simulink library "Linkage"  (R2025b)
settings: Solver=VariableStepAuto  StartTime=0.0  StopTime=10.0  RelTol=1e-3
undefined symbols (not defined in the file): Axle1D, AxleIn, Chassis, Init, RaceFix, RaceSpin, Vehicle, Visual, X, Y, Z
libraries: sm_lib x940, nesl_utility x136, fl_lib x6, Linkage_Systems x2, SteeringWheel x2, Linkage_Decoupled x2, AntiRollBar_Systems x1, Steer_Rack_None x1, Steer_Rack_WheelDrivenRack1UJoint x1
(part 4 of 25)

== system Linkage/Susp/Linkage Decoupled/RollHeave Decouple/HP Heave L ==
  note: Shock point is not mirrored to permit independent point definition on left and right sides.
  note: Aligns pivot axis with vector normal to three hardpoints.
  Revolute Pivot : sm_lib/Joints/Revolute Joint  JointMode=Normal  CompositeWrenchDir=FollowerOnBase  CompositeWrenchFrame=BaseFrame  SenseConstraintForce=off  SenseConstraintTorque=off  SenseTotalForce=off  SenseTotalTorque=off  PositionTargetSpecify=off  PositionTargetPriority=Low  PositionTargetValue=0  PositionTargetValueUnits=deg  VelocityTargetSpecify=off  VelocityTargetPriority=High  VelocityTargetValue=0  VelocityTargetValueUnits=deg/s  EquilibriumPosition=0  EquilibriumPositionUnits=deg  SpringStiffness=0  SpringStiffnessUnits=N*m/deg  DampingCoefficient=0  DampingCoefficientUnits=N*m/(deg/s)  LowerLimitSpecify=off  LowerLimitBound=-90  LowerLimitBoundUnits=deg  LowerLimitStiffness=1e4  LowerLimitStiffnessUnits=N*m/deg  LowerLimitDamping=10  LowerLimitDampingUnits=N*m/(deg/s)  LowerLimitTransitionRegionWidth=0.1  LowerLimitTransitionRegionWidthUnits=deg  UpperLimitSpecify=off  UpperLimitBound=90  UpperLimitBoundUnits=deg  UpperLimitStiffness=1e4  UpperLimitStiffnessUnits=N*m/deg  UpperLimitDamping=10  UpperLimitDampingUnits=N*m/(deg/s)  UpperLimitTransitionRegionWidth=0.1  UpperLimitTransitionRegionWidthUnits=deg  TorqueActuationMode=NoTorque  MotionActuationMode=ComputedMotion  SensePosition=on  SenseVelocity=off  SenseAcceleration=off  SenseTorqueForce=off  SenseLowerLimitTorqueForce=off  SenseUpperLimitTorqueForce=off
  Transform Align Axis B : Subsystem  mask(Transform Align Axis Three Points){pt1=hp_bcr_pivot.*rhs_hp, pt2=hp_pushrod_in.*rhs_hp, pt3=hp_bcr_shock, popup_f_axis=+Z}
      mask prompts: pt1 "Point 1 [xyz] (m)"; pt2 "Point 2 [xyz] (m)"; pt3 "Point 3 [xyz] (m)"; popup_f_axis "Axis of F Frame to Aim at Target"
      mask help: Transforms a frame to aim a selected axis along a normal to a plane defined by 3 points. All points must be defined relative to the same reference frame. Normal to the plane is defined as cross (HP1 -> HP3, HP1->HP2).
      mask init:
      | switch popup_f_axis
      |     case 1, vec = [ 1  0  0];
      |     case 2, vec = [ 0  1  0];
      |     case 3, vec = [ 0  0  1];
      |     case 4, vec = [-1  0  0];
      |     case 5, vec = [ 0 -1  0];
      |     case 6, vec = [ 0  0 -1];
      | end
      | 
      | % Unit vectors 
      | uvec1 = (pt3-pt1)/norm(pt3-pt1);
      | uvec2 = (pt2-pt1)/norm(pt2-pt1);
      | 
      | nvec = cross(uvec1,uvec2);
      | unvec = nvec/norm(nvec);
      | 
      | % Force nvec to point along +z
      | %if(unvec(3)<0)
      | %    unvec = -unvec;
      | %end
      | rotaxis = cross(vec,unvec);
      | 
      | if (norm(rotaxis)==0)
      |     if (sum(uvec1==0)==3 || sum(uvec2==0)==3)  % hps collocated
      |         rotangle = 0; 
      |     elseif ((sum(uvec1+uvec2)==0) ...  % vectors antiparallel    
      |             || (sum(vec+unvec))==0)    % vec and unvec antiparallel
      |         rotangle = pi;
      |         rotaxis = circshift(vec,1);
      |     else                       % vectors parallel
      |         rotangle = 0;          
      |     end
      | else
      |     rotangle = acos(dot(vec,unvec));
      |     %rotangle = acos(dot(vec,(hp_t-hp_b)/norm((hp_t-hp_b))))
      | end
      mask TypeOptions popup_f_axis: +X | +Y | +Z | -X | -Y | -Z
      mask Display: image('sm_car_transform_align_axis_three_points.png')
  Transform Align Axis F : Subsystem  mask(Transform Align Axis Three Points){pt1=hp_bcr_pivot.*rhs_hp, pt2=hp_pushrod_in.*rhs_hp, pt3=hp_bcr_shock, popup_f_axis=+Z}
      mask prompts: pt1 "Point 1 [xyz] (m)"; pt2 "Point 2 [xyz] (m)"; pt3 "Point 3 [xyz] (m)"; popup_f_axis "Axis of F Frame to Aim at Target"
      mask help: Transforms a frame to aim a selected axis along a normal to a plane defined by 3 points. All points must be defined relative to the same reference frame. Normal to the plane is defined as cross (HP1 -> HP3, HP1->HP2).
      mask init: same as Linkage/Susp/Linkage Decoupled/RollHeave Decouple/HP Heave L/Transform Align Axis B
      mask TypeOptions popup_f_axis: +X | +Y | +Z | -X | -Y | -Z
      mask Display: image('sm_car_transform_align_axis_three_points.png')
  F : PMIOPort  Side=Right
  B : PMIOPort  Port=2  Side=Left
  q : PMIOPort  Port=3  Side=Right
  connections:
  Transform Align Axis B/LConn1 -- B/RConn1
  Transform Align Axis F/RConn1 -- Revolute Pivot/RConn1
  Revolute Pivot/LConn1 -- Transform Align Axis B/RConn1
  Transform Align Axis F/LConn1 -- F/RConn1
  q/RConn1 -- Revolute Pivot/RConn2

== system Linkage/Susp/Linkage Decoupled/RollHeave Decouple/HP HeaveR ==
  note: Shock point is not mirrored to permit independent point definition on left and right sides.
  note: Aligns pivot axis with vector normal to three hardpoints.
  Revolute Pivot : sm_lib/Joints/Revolute Joint  JointMode=Normal  CompositeWrenchDir=FollowerOnBase  CompositeWrenchFrame=BaseFrame  SenseConstraintForce=off  SenseConstraintTorque=off  SenseTotalForce=off  SenseTotalTorque=off  PositionTargetSpecify=off  PositionTargetPriority=Low  PositionTargetValue=0  PositionTargetValueUnits=deg  VelocityTargetSpecify=off  VelocityTargetPriority=High  VelocityTargetValue=0  VelocityTargetValueUnits=deg/s  EquilibriumPosition=0  EquilibriumPositionUnits=deg  SpringStiffness=0  SpringStiffnessUnits=N*m/deg  DampingCoefficient=0  DampingCoefficientUnits=N*m/(deg/s)  LowerLimitSpecify=off  LowerLimitBound=-90  LowerLimitBoundUnits=deg  LowerLimitStiffness=1e4  LowerLimitStiffnessUnits=N*m/deg  LowerLimitDamping=10  LowerLimitDampingUnits=N*m/(deg/s)  LowerLimitTransitionRegionWidth=0.1  LowerLimitTransitionRegionWidthUnits=deg  UpperLimitSpecify=off  UpperLimitBound=90  UpperLimitBoundUnits=deg  UpperLimitStiffness=1e4  UpperLimitStiffnessUnits=N*m/deg  UpperLimitDamping=10  UpperLimitDampingUnits=N*m/(deg/s)  UpperLimitTransitionRegionWidth=0.1  UpperLimitTransitionRegionWidthUnits=deg  TorqueActuationMode=NoTorque  MotionActuationMode=ComputedMotion  SensePosition=on  SenseVelocity=off  SenseAcceleration=off  SenseTorqueForce=off  SenseLowerLimitTorqueForce=off  SenseUpperLimitTorqueForce=off
  Transform Align Axis B : Subsystem  mask(Transform Align Axis Three Points){pt1=hp_bcr_pivot.*rhs_hp, pt2=hp_pushrod_in.*rhs_hp, pt3=hp_bcr_shock, popup_f_axis=+Z}
      mask prompts: pt1 "Point 1 [xyz] (m)"; pt2 "Point 2 [xyz] (m)"; pt3 "Point 3 [xyz] (m)"; popup_f_axis "Axis of F Frame to Aim at Target"
      mask help: Transforms a frame to aim a selected axis along a normal to a plane defined by 3 points. All points must be defined relative to the same reference frame. Normal to the plane is defined as cross (HP1 -> HP3, HP1->HP2).
      mask init: same as Linkage/Susp/Linkage Decoupled/RollHeave Decouple/HP Heave L/Transform Align Axis B
      mask TypeOptions popup_f_axis: +X | +Y | +Z | -X | -Y | -Z
      mask Display: image('sm_car_transform_align_axis_three_points.png')
  Transform Align Axis F : Subsystem  mask(Transform Align Axis Three Points){pt1=hp_bcr_pivot.*rhs_hp, pt2=hp_pushrod_in.*rhs_hp, pt3=hp_bcr_shock, popup_f_axis=+Z}
      mask prompts: pt1 "Point 1 [xyz] (m)"; pt2 "Point 2 [xyz] (m)"; pt3 "Point 3 [xyz] (m)"; popup_f_axis "Axis of F Frame to Aim at Target"
      mask help: Transforms a frame to aim a selected axis along a normal to a plane defined by 3 points. All points must be defined relative to the same reference frame. Normal to the plane is defined as cross (HP1 -> HP3, HP1->HP2).
      mask init: same as Linkage/Susp/Linkage Decoupled/RollHeave Decouple/HP Heave L/Transform Align Axis B
      mask TypeOptions popup_f_axis: +X | +Y | +Z | -X | -Y | -Z
      mask Display: image('sm_car_transform_align_axis_three_points.png')
  F : PMIOPort  Side=Right
  B : PMIOPort  Port=2  Side=Left
  q : PMIOPort  Port=3  Side=Right
  connections:
  Transform Align Axis F/LConn1 -- F/RConn1
  Revolute Pivot/LConn1 -- Transform Align Axis B/RConn1
  Transform Align Axis F/RConn1 -- Revolute Pivot/RConn1
  Transform Align Axis B/LConn1 -- B/RConn1
  q/RConn1 -- Revolute Pivot/RConn2

== system Linkage/Susp/Linkage Decoupled/RollHeave Decouple/HP Roll L ==
  note: Shock point is not mirrored to permit independent point definition on left and right sides.
  note: Aligns pivot axis with vector normal to three hardpoints.
  Revolute Pivot : sm_lib/Joints/Revolute Joint  JointMode=Normal  CompositeWrenchDir=FollowerOnBase  CompositeWrenchFrame=BaseFrame  SenseConstraintForce=off  SenseConstraintTorque=off  SenseTotalForce=off  SenseTotalTorque=off  PositionTargetSpecify=off  PositionTargetPriority=Low  PositionTargetValue=0  PositionTargetValueUnits=deg  VelocityTargetSpecify=off  VelocityTargetPriority=High  VelocityTargetValue=0  VelocityTargetValueUnits=deg/s  EquilibriumPosition=0  EquilibriumPositionUnits=deg  SpringStiffness=0  SpringStiffnessUnits=N*m/deg  DampingCoefficient=0  DampingCoefficientUnits=N*m/(deg/s)  LowerLimitSpecify=off  LowerLimitBound=-90  LowerLimitBoundUnits=deg  LowerLimitStiffness=1e4  LowerLimitStiffnessUnits=N*m/deg  LowerLimitDamping=10  LowerLimitDampingUnits=N*m/(deg/s)  LowerLimitTransitionRegionWidth=0.1  LowerLimitTransitionRegionWidthUnits=deg  UpperLimitSpecify=off  UpperLimitBound=90  UpperLimitBoundUnits=deg  UpperLimitStiffness=1e4  UpperLimitStiffnessUnits=N*m/deg  UpperLimitDamping=10  UpperLimitDampingUnits=N*m/(deg/s)  UpperLimitTransitionRegionWidth=0.1  UpperLimitTransitionRegionWidthUnits=deg  TorqueActuationMode=NoTorque  MotionActuationMode=ComputedMotion  SensePosition=on  SenseVelocity=off  SenseAcceleration=off  SenseTorqueForce=off  SenseLowerLimitTorqueForce=off  SenseUpperLimitTorqueForce=off
  Transform Align Axis B : Subsystem  mask(Transform Align Axis Three Points){pt1=hp_bcr_pivot.*rhs_hp, pt2=hp_pushrod_in.*rhs_hp, pt3=hp_bcr_shock, popup_f_axis=+Z}
      mask prompts: pt1 "Point 1 [xyz] (m)"; pt2 "Point 2 [xyz] (m)"; pt3 "Point 3 [xyz] (m)"; popup_f_axis "Axis of F Frame to Aim at Target"
      mask help: Transforms a frame to aim a selected axis along a normal to a plane defined by 3 points. All points must be defined relative to the same reference frame. Normal to the plane is defined as cross (HP1 -> HP3, HP1->HP2).
      mask init: same as Linkage/Susp/Linkage Decoupled/RollHeave Decouple/HP Heave L/Transform Align Axis B
      mask TypeOptions popup_f_axis: +X | +Y | +Z | -X | -Y | -Z
      mask Display: image('sm_car_transform_align_axis_three_points.png')
  Transform Align Axis F : Subsystem  mask(Transform Align Axis Three Points){pt1=hp_bcr_pivot.*rhs_hp, pt2=hp_pushrod_in.*rhs_hp, pt3=hp_bcr_shock, popup_f_axis=+Z}
      mask prompts: pt1 "Point 1 [xyz] (m)"; pt2 "Point 2 [xyz] (m)"; pt3 "Point 3 [xyz] (m)"; popup_f_axis "Axis of F Frame to Aim at Target"
      mask help: Transforms a frame to aim a selected axis along a normal to a plane defined by 3 points. All points must be defined relative to the same reference frame. Normal to the plane is defined as cross (HP1 -> HP3, HP1->HP2).
      mask init: same as Linkage/Susp/Linkage Decoupled/RollHeave Decouple/HP Heave L/Transform Align Axis B
      mask TypeOptions popup_f_axis: +X | +Y | +Z | -X | -Y | -Z
      mask Display: image('sm_car_transform_align_axis_three_points.png')
  F : PMIOPort  Side=Right
  B : PMIOPort  Port=2  Side=Left
  q : PMIOPort  Port=3  Side=Right
  connections:
  Transform Align Axis F/LConn1 -- F/RConn1
  Revolute Pivot/LConn1 -- Transform Align Axis B/RConn1
  Transform Align Axis F/RConn1 -- Revolute Pivot/RConn1
  Transform Align Axis B/LConn1 -- B/RConn1
  q/RConn1 -- Revolute Pivot/RConn2

== system Linkage/Susp/Linkage Decoupled/RollHeave Decouple/HP Roll R ==
  note: Shock point is not mirrored to permit independent point definition on left and right sides.
  note: Aligns pivot axis with vector normal to three hardpoints.
  Revolute Pivot : sm_lib/Joints/Revolute Joint  JointMode=Normal  CompositeWrenchDir=FollowerOnBase  CompositeWrenchFrame=BaseFrame  SenseConstraintForce=off  SenseConstraintTorque=off  SenseTotalForce=off  SenseTotalTorque=off  PositionTargetSpecify=off  PositionTargetPriority=Low  PositionTargetValue=0  PositionTargetValueUnits=deg  VelocityTargetSpecify=off  VelocityTargetPriority=High  VelocityTargetValue=0  VelocityTargetValueUnits=deg/s  EquilibriumPosition=0  EquilibriumPositionUnits=deg  SpringStiffness=0  SpringStiffnessUnits=N*m/deg  DampingCoefficient=0  DampingCoefficientUnits=N*m/(deg/s)  LowerLimitSpecify=off  LowerLimitBound=-90  LowerLimitBoundUnits=deg  LowerLimitStiffness=1e4  LowerLimitStiffnessUnits=N*m/deg  LowerLimitDamping=10  LowerLimitDampingUnits=N*m/(deg/s)  LowerLimitTransitionRegionWidth=0.1  LowerLimitTransitionRegionWidthUnits=deg  UpperLimitSpecify=off  UpperLimitBound=90  UpperLimitBoundUnits=deg  UpperLimitStiffness=1e4  UpperLimitStiffnessUnits=N*m/deg  UpperLimitDamping=10  UpperLimitDampingUnits=N*m/(deg/s)  UpperLimitTransitionRegionWidth=0.1  UpperLimitTransitionRegionWidthUnits=deg  TorqueActuationMode=NoTorque  MotionActuationMode=ComputedMotion  SensePosition=on  SenseVelocity=off  SenseAcceleration=off  SenseTorqueForce=off  SenseLowerLimitTorqueForce=off  SenseUpperLimitTorqueForce=off
  Transform Align Axis B : Subsystem  mask(Transform Align Axis Three Points){pt1=hp_bcr_pivot.*rhs_hp, pt2=hp_pushrod_in.*rhs_hp, pt3=hp_bcr_shock, popup_f_axis=+Z}
      mask prompts: pt1 "Point 1 [xyz] (m)"; pt2 "Point 2 [xyz] (m)"; pt3 "Point 3 [xyz] (m)"; popup_f_axis "Axis of F Frame to Aim at Target"
      mask help: Transforms a frame to aim a selected axis along a normal to a plane defined by 3 points. All points must be defined relative to the same reference frame. Normal to the plane is defined as cross (HP1 -> HP3, HP1->HP2).
      mask init: same as Linkage/Susp/Linkage Decoupled/RollHeave Decouple/HP Heave L/Transform Align Axis B
      mask TypeOptions popup_f_axis: +X | +Y | +Z | -X | -Y | -Z
      mask Display: image('sm_car_transform_align_axis_three_points.png')
  Transform Align Axis F : Subsystem  mask(Transform Align Axis Three Points){pt1=hp_bcr_pivot.*rhs_hp, pt2=hp_pushrod_in.*rhs_hp, pt3=hp_bcr_shock, popup_f_axis=+Z}
      mask prompts: pt1 "Point 1 [xyz] (m)"; pt2 "Point 2 [xyz] (m)"; pt3 "Point 3 [xyz] (m)"; popup_f_axis "Axis of F Frame to Aim at Target"
      mask help: Transforms a frame to aim a selected axis along a normal to a plane defined by 3 points. All points must be defined relative to the same reference frame. Normal to the plane is defined as cross (HP1 -> HP3, HP1->HP2).
      mask init: same as Linkage/Susp/Linkage Decoupled/RollHeave Decouple/HP Heave L/Transform Align Axis B
      mask TypeOptions popup_f_axis: +X | +Y | +Z | -X | -Y | -Z
      mask Display: image('sm_car_transform_align_axis_three_points.png')
  F : PMIOPort  Side=Right
  B : PMIOPort  Port=2  Side=Left
  q : PMIOPort  Port=3  Side=Right
  connections:
  Transform Align Axis B/LConn1 -- B/RConn1
  Transform Align Axis F/RConn1 -- Revolute Pivot/RConn1
  Revolute Pivot/LConn1 -- Transform Align Axis B/RConn1
  Transform Align Axis F/LConn1 -- F/RConn1
  q/RConn1 -- Revolute Pivot/RConn2

== system Linkage/Susp/Linkage Decoupled/RollHeave Decouple/Shock Heave ==
  Cylinder : Subsystem
  MTRef : fl_lib/Mechanical/Translational Elements/Mechanical Translational Reference
  PS-Simulink Converter : nesl_utility/PS-Simulink Converter  PhysicalDomain=network_engine_domain  SubClassName=ps_output  LeftPortType=input  RightPortType=output  PseudoPeriodic=off  Frequencies=[]  VectorFormat=1-D array  Unit=1  AffineConversion=off
  Piston : Subsystem
  Prismatic Spring : sm_lib/Joints/Prismatic Joint  JointMode=Normal  CompositeWrenchDir=FollowerOnBase  CompositeWrenchFrame=BaseFrame  SenseConstraintForce=off  SenseConstraintTorque=off  SenseTotalForce=off  SenseTotalTorque=off  PositionTargetSpecify=on  PositionTargetPriority=High  PositionTargetValue=init_spr_len  PositionTargetValueUnits=m  VelocityTargetSpecify=off  VelocityTargetPriority=High  VelocityTargetValue=0  VelocityTargetValueUnits=m/s  EquilibriumPosition=0  EquilibriumPositionUnits=m  SpringStiffness=0  SpringStiffnessUnits=N/m  DampingCoefficient=0.01  DampingCoefficientUnits=N/(m/s)  LowerLimitSpecify=off  LowerLimitBound=-1  LowerLimitBoundUnits=m  LowerLimitStiffness=1e6  LowerLimitStiffnessUnits=N/m  LowerLimitDamping=1e3  LowerLimitDampingUnits=N/(m/s)  LowerLimitTransitionRegionWidth=1e-4  LowerLimitTransitionRegionWidthUnits=m  UpperLimitSpecify=off  UpperLimitBound=1  UpperLimitBoundUnits=m  UpperLimitStiffness=1e6  UpperLimitStiffnessUnits=N/m  UpperLimitDamping=1e3  UpperLimitDampingUnits=N/(m/s)  UpperLimitTransitionRegionWidth=1e-4  UpperLimitTransitionRegionWidthUnits=m  TorqueActuationMode=InputTorque  MotionActuationMode=ComputedMotion  SensePosition=on  SenseVelocity=on  SenseAcceleration=off  SenseTorqueForce=off  SenseLowerLimitTorqueForce=off  SenseUpperLimitTorqueForce=off
  Translational Simscape Intf : Subsystem
  Vis HP L : sm_lib/Body Elements/Spherical Solid  SphereRadius=size_conn_shock  SphereRadiusUnits=m  ExportEntireGeometry=off  InertiaType=PointMass  BasedOnType=Density  Density=0  DensityUnits=kg/m^3  Mass=0  MassUnits=kg  CenterOfMass=[0 0 0]  CenterOfMassUnits=m  MomentsOfInertia=[1 1 1]  MomentsOfInertiaUnits=kg*m^2  ProductsOfInertia=[0 0 0]  ProductsOfInertiaUnits=kg*m^2  GraphicType=FromGeometry  MarkerShape=Sphere  MarkerSize=10  GraphicVisPropType=SimpleVisualProperties  GraphicDiffuseColor=clr_conn_shock  GraphicOpacity=opc_conn_shock  GraphicSpecularColor=[0.5 0.5 0.5 1.0]  GraphicAmbientColor=[0.15 0.15 0.15 1.0]  GraphicEmissiveColor=[0.0 0.0 0.0 1.0]  GraphicShininess=75  DoExposeReferenceFrame=on  SerializedFrames=<Frames/>
  Vis HP U : sm_lib/Body Elements/Spherical Solid  SphereRadius=size_conn_shock  SphereRadiusUnits=m  ExportEntireGeometry=off  InertiaType=PointMass  BasedOnType=Density  Density=0  DensityUnits=kg/m^3  Mass=0  MassUnits=kg  CenterOfMass=[0 0 0]  CenterOfMassUnits=m  MomentsOfInertia=[1 1 1]  MomentsOfInertiaUnits=kg*m^2  ProductsOfInertia=[0 0 0]  ProductsOfInertiaUnits=kg*m^2  GraphicType=FromGeometry  MarkerShape=Sphere  MarkerSize=10  GraphicVisPropType=SimpleVisualProperties  GraphicDiffuseColor=clr_conn_shock  GraphicOpacity=opc_conn_shock  GraphicSpecularColor=[0.5 0.5 0.5 1.0]  GraphicAmbientColor=[0.15 0.15 0.15 1.0]  GraphicEmissiveColor=[0.0 0.0 0.0 1.0]  GraphicShininess=75  DoExposeReferenceFrame=on  SerializedFrames=<Frames/>
  R : PMIOPort  Side=Right
  U : PMIOPort  Port=2  Side=Right
  L : PMIOPort  Port=3  Side=Left
  Out Bus Element : Outport  VectorParamsAs1DForOutWhenUnconnected=off  PortName=m  Element=x
  wires:
  PS-Simulink Converter/1 -> Out Bus Element/1
  connections:
  PS-Simulink Converter/LConn1 -- Prismatic Spring/RConn2
  Vis HP L/RConn1 -- Cylinder/LConn1 -- Prismatic Spring/LConn1 -- L/RConn1
  Translational Simscape Intf/LConn1 -- Prismatic Spring/LConn2
  Translational Simscape Intf/RConn1 -- Prismatic Spring/RConn3
  Vis HP U/RConn1 -- U/RConn1 -- Prismatic Spring/RConn1 -- Piston/RConn1
  MTRef/LConn1 -- Translational Simscape Intf/LConn2
  R/RConn1 -- Translational Simscape Intf/RConn2

== system Linkage/Susp/Linkage Decoupled/RollHeave Decouple/Shock Roll ==
  Cylinder : Subsystem
  MTRef : fl_lib/Mechanical/Translational Elements/Mechanical Translational Reference
  PS-Simulink Converter : nesl_utility/PS-Simulink Converter  PhysicalDomain=network_engine_domain  SubClassName=ps_output  LeftPortType=input  RightPortType=output  PseudoPeriodic=off  Frequencies=[]  VectorFormat=1-D array  Unit=1  AffineConversion=off
  Piston : Subsystem
  Prismatic Spring : sm_lib/Joints/Prismatic Joint  JointMode=Normal  CompositeWrenchDir=FollowerOnBase  CompositeWrenchFrame=BaseFrame  SenseConstraintForce=off  SenseConstraintTorque=off  SenseTotalForce=off  SenseTotalTorque=off  PositionTargetSpecify=on  PositionTargetPriority=High  PositionTargetValue=init_spr_len  PositionTargetValueUnits=m  VelocityTargetSpecify=off  VelocityTargetPriority=High  VelocityTargetValue=0  VelocityTargetValueUnits=m/s  EquilibriumPosition=0  EquilibriumPositionUnits=m  SpringStiffness=0  SpringStiffnessUnits=N/m  DampingCoefficient=0.01  DampingCoefficientUnits=N/(m/s)  LowerLimitSpecify=off  LowerLimitBound=-1  LowerLimitBoundUnits=m  LowerLimitStiffness=1e6  LowerLimitStiffnessUnits=N/m  LowerLimitDamping=1e3  LowerLimitDampingUnits=N/(m/s)  LowerLimitTransitionRegionWidth=1e-4  LowerLimitTransitionRegionWidthUnits=m  UpperLimitSpecify=off  UpperLimitBound=1  UpperLimitBoundUnits=m  UpperLimitStiffness=1e6  UpperLimitStiffnessUnits=N/m  UpperLimitDamping=1e3  UpperLimitDampingUnits=N/(m/s)  UpperLimitTransitionRegionWidth=1e-4  UpperLimitTransitionRegionWidthUnits=m  TorqueActuationMode=InputTorque  MotionActuationMode=ComputedMotion  SensePosition=on  SenseVelocity=on  SenseAcceleration=off  SenseTorqueForce=off  SenseLowerLimitTorqueForce=off  SenseUpperLimitTorqueForce=off
  Translational Simscape Intf : Subsystem
  Vis HP L : sm_lib/Body Elements/Spherical Solid  SphereRadius=size_conn_shock  SphereRadiusUnits=m  ExportEntireGeometry=off  InertiaType=PointMass  BasedOnType=Density  Density=0  DensityUnits=kg/m^3  Mass=0  MassUnits=kg  CenterOfMass=[0 0 0]  CenterOfMassUnits=m  MomentsOfInertia=[1 1 1]  MomentsOfInertiaUnits=kg*m^2  ProductsOfInertia=[0 0 0]  ProductsOfInertiaUnits=kg*m^2  GraphicType=FromGeometry  MarkerShape=Sphere  MarkerSize=10  GraphicVisPropType=SimpleVisualProperties  GraphicDiffuseColor=clr_conn_shock  GraphicOpacity=opc_conn_shock  GraphicSpecularColor=[0.5 0.5 0.5 1.0]  GraphicAmbientColor=[0.15 0.15 0.15 1.0]  GraphicEmissiveColor=[0.0 0.0 0.0 1.0]  GraphicShininess=75  DoExposeReferenceFrame=on  SerializedFrames=<Frames/>
  Vis HP U : sm_lib/Body Elements/Spherical Solid  SphereRadius=size_conn_shock  SphereRadiusUnits=m  ExportEntireGeometry=off  InertiaType=PointMass  BasedOnType=Density  Density=0  DensityUnits=kg/m^3  Mass=0  MassUnits=kg  CenterOfMass=[0 0 0]  CenterOfMassUnits=m  MomentsOfInertia=[1 1 1]  MomentsOfInertiaUnits=kg*m^2  ProductsOfInertia=[0 0 0]  ProductsOfInertiaUnits=kg*m^2  GraphicType=FromGeometry  MarkerShape=Sphere  MarkerSize=10  GraphicVisPropType=SimpleVisualProperties  GraphicDiffuseColor=clr_conn_shock  GraphicOpacity=opc_conn_shock  GraphicSpecularColor=[0.5 0.5 0.5 1.0]  GraphicAmbientColor=[0.15 0.15 0.15 1.0]  GraphicEmissiveColor=[0.0 0.0 0.0 1.0]  GraphicShininess=75  DoExposeReferenceFrame=on  SerializedFrames=<Frames/>
  R : PMIOPort  Side=Right
  U : PMIOPort  Port=2  Side=Right
  L : PMIOPort  Port=3  Side=Left
  Out Bus Element : Outport  VectorParamsAs1DForOutWhenUnconnected=off  PortName=m  Element=x
  wires:
  PS-Simulink Converter/1 -> Out Bus Element/1
  connections:
  PS-Simulink Converter/LConn1 -- Prismatic Spring/RConn2
  Vis HP L/RConn1 -- Cylinder/LConn1 -- Prismatic Spring/LConn1 -- L/RConn1
  Translational Simscape Intf/LConn1 -- Prismatic Spring/LConn2
  Translational Simscape Intf/RConn1 -- Prismatic Spring/RConn3
  Vis HP U/RConn1 -- U/RConn1 -- Prismatic Spring/RConn1 -- Piston/RConn1
  MTRef/LConn1 -- Translational Simscape Intf/LConn2
  R/RConn1 -- Translational Simscape Intf/RConn2

== system Linkage/Susp/Linkage Decoupled/RollHeave Decouple/Transform Align Axis 2P HeaveL ==
  Transform : sm_lib/Frames and Transforms/Rigid Transform  RotationMethod=ArbitraryAxis  FollAlignAxisA=+X  BaseAlignAxisA=+Y  FollAlignAxisB=+Y  BaseAlignAxisB=+Z  RotationStandardAxis=+Z  RotationAngle=rotangle  RotationAngleUnits=rad  RotationArbitraryAxis=rotaxis  RotationSequenceAxes=FollowerAxes  RotationSequence=XYX  RotationSequenceAngles=[0 0 0]  RotationSequenceAnglesUnits=deg  RotationMatrix=[1 0 0; 0 1 0; 0 0 1]  Quaternion=[1 0 0 0]  TranslationMethod=None  TranslationCartesianOffset=[0 0 0]  TranslationCartesianOffsetUnits=m  TranslationStandardAxis=+Z  TranslationStandardOffset=0  TranslationStandardOffsetUnits=m  TranslationROffset=0  TranslationROffsetUnits=m  TranslationThetaOffset=0  TranslationThetaOffsetUnits=deg  TranslationZOffset=0  TranslationZOffsetUnits=m
  B : PMIOPort  Side=Left
  F : PMIOPort  Port=2  Side=Right
  connections:
  Transform/LConn1 -- B/RConn1
  Transform/RConn1 -- F/RConn1

== system Linkage/Susp/Linkage Decoupled/RollHeave Decouple/Transform Align Axis 2P HeaveR ==
  Transform : sm_lib/Frames and Transforms/Rigid Transform  RotationMethod=ArbitraryAxis  FollAlignAxisA=+X  BaseAlignAxisA=+Y  FollAlignAxisB=+Y  BaseAlignAxisB=+Z  RotationStandardAxis=+Z  RotationAngle=rotangle  RotationAngleUnits=rad  RotationArbitraryAxis=rotaxis  RotationSequenceAxes=FollowerAxes  RotationSequence=XYX  RotationSequenceAngles=[0 0 0]  RotationSequenceAnglesUnits=deg  RotationMatrix=[1 0 0; 0 1 0; 0 0 1]  Quaternion=[1 0 0 0]  TranslationMethod=None  TranslationCartesianOffset=[0 0 0]  TranslationCartesianOffsetUnits=m  TranslationStandardAxis=+Z  TranslationStandardOffset=0  TranslationStandardOffsetUnits=m  TranslationROffset=0  TranslationROffsetUnits=m  TranslationThetaOffset=0  TranslationThetaOffsetUnits=deg  TranslationZOffset=0  TranslationZOffsetUnits=m
  B : PMIOPort  Side=Left
  F : PMIOPort  Port=2  Side=Right
  connections:
  Transform/LConn1 -- B/RConn1
  Transform/RConn1 -- F/RConn1

== system Linkage/Susp/Linkage Decoupled/RollHeave Decouple/Transform Align Axis 2P RollL ==
  Transform : sm_lib/Frames and Transforms/Rigid Transform  RotationMethod=ArbitraryAxis  FollAlignAxisA=+X  BaseAlignAxisA=+Y  FollAlignAxisB=+Y  BaseAlignAxisB=+Z  RotationStandardAxis=+Z  RotationAngle=rotangle  RotationAngleUnits=rad  RotationArbitraryAxis=rotaxis  RotationSequenceAxes=FollowerAxes  RotationSequence=XYX  RotationSequenceAngles=[0 0 0]  RotationSequenceAnglesUnits=deg  RotationMatrix=[1 0 0; 0 1 0; 0 0 1]  Quaternion=[1 0 0 0]  TranslationMethod=None  TranslationCartesianOffset=[0 0 0]  TranslationCartesianOffsetUnits=m  TranslationStandardAxis=+Z  TranslationStandardOffset=0  TranslationStandardOffsetUnits=m  TranslationROffset=0  TranslationROffsetUnits=m  TranslationThetaOffset=0  TranslationThetaOffsetUnits=deg  TranslationZOffset=0  TranslationZOffsetUnits=m
  B : PMIOPort  Side=Left
  F : PMIOPort  Port=2  Side=Right
  connections:
  Transform/LConn1 -- B/RConn1
  Transform/RConn1 -- F/RConn1

== system Linkage/Susp/Linkage Decoupled/RollHeave Decouple/Transform Align Axis 2P RollR ==
  Transform : sm_lib/Frames and Transforms/Rigid Transform  RotationMethod=ArbitraryAxis  FollAlignAxisA=+X  BaseAlignAxisA=+Y  FollAlignAxisB=+Y  BaseAlignAxisB=+Z  RotationStandardAxis=+Z  RotationAngle=rotangle  RotationAngleUnits=rad  RotationArbitraryAxis=rotaxis  RotationSequenceAxes=FollowerAxes  RotationSequence=XYX  RotationSequenceAngles=[0 0 0]  RotationSequenceAnglesUnits=deg  RotationMatrix=[1 0 0; 0 1 0; 0 0 1]  Quaternion=[1 0 0 0]  TranslationMethod=None  TranslationCartesianOffset=[0 0 0]  TranslationCartesianOffsetUnits=m  TranslationStandardAxis=+Z  TranslationStandardOffset=0  TranslationStandardOffsetUnits=m  TranslationROffset=0  TranslationROffsetUnits=m  TranslationThetaOffset=0  TranslationThetaOffsetUnits=deg  TranslationZOffset=0  TranslationZOffsetUnits=m
  B : PMIOPort  Side=Left
  F : PMIOPort  Port=2  Side=Right
  connections:
  Transform/LConn1 -- B/RConn1
  Transform/RConn1 -- F/RConn1

== system Linkage/Susp/Linkage Decoupled/Steer/None ==
  In Bus Element1 : Inport  PortName=DrvBus  Element=aSteerWheel
  In Bus Element2 : Inport  Port=2  PortName=CtrlBus
  Body Sensor : Subsystem  mask{offset_body_sensor=Vehicle.Chassis.Body.sCG.Value}
      mask prompts: offset_body_sensor "Sensor Frame Offset [x y z] (m)"
  Constant : Constant  Value=0
  Constant1 : Constant  Value=0
  Constant2 : Constant  Value=0
  Terminator : Terminator
  Terminator1 : Terminator
  rodL : PMIOPort  Side=Right
  ref : PMIOPort  Port=2  Side=Right
  rodR : PMIOPort  Port=3  Side=Right
  Out Bus Element : Outport  VectorParamsAs1DForOutWhenUnconnected=off  PortName=meas  Element=FRack
  Out Bus Element1 : Outport  VectorParamsAs1DForOutWhenUnconnected=off  PortName=meas  Element=xRack
  Out Bus Element2 : Outport  VectorParamsAs1DForOutWhenUnconnected=off  PortName=meas  Element=aWheel
  Out Bus Element3 : Outport  VectorParamsAs1DForOutWhenUnconnected=off  PortName=meas  Element=Driver
  wires:
  Body Sensor/1(Body) -> Out Bus Element3/1
  Constant2/1 -> Out Bus Element2/1
  In Bus Element2/1 -> Terminator1/1
  Constant1/1 -> Out Bus Element/1
  Constant/1 -> Out Bus Element1/1
  In Bus Element1/1 -> Terminator/1
  connections:
  rodR/RConn1 -- ref/RConn1 -- Body Sensor/LConn1 -- rodL/RConn1

== system Linkage/Susp/Linkage Decoupled/Steer/Rack ==
  In Bus Element1 : Inport  PortName=DrvBus  Element=aSteerWheel
  In Bus Element2 : Inport  Port=2  PortName=CtrlBus
  In Bus Element : Inport  Port=2  PortName=CtrlBus  Element=aSteerWheel
  Body Sensor : Subsystem  mask{offset_body_sensor=Vehicle.Chassis.Body.sCG.Value}
      mask prompts: offset_body_sensor "Sensor Frame Offset [x y z] (m)"
  Constant : Constant  Value=0
  PS-SL fRack : nesl_utility/PS-Simulink Converter  PhysicalDomain=network_engine_domain  SubClassName=ps_output  LeftPortType=input  RightPortType=output  PseudoPeriodic=off  Frequencies=[]  VectorFormat=1-D array  Unit=1  AffineConversion=off
  PS-SL xRack : nesl_utility/PS-Simulink Converter  PhysicalDomain=network_engine_domain  SubClassName=ps_output  LeftPortType=input  RightPortType=output  PseudoPeriodic=off  Frequencies=[]  VectorFormat=1-D array  Unit=1  AffineConversion=off
  Physical Signal : nesl_utility/Simulink-PS Converter  PhysicalDomain=network_engine_domain  SubClassName=ps_input  LeftPortType=input  RightPortType=output  PseudoPeriodic=off  Frequencies=[]  NoiseDistribution=none  NoiseParameters=[]  Unit=m  AffineConversion=off  FilteringAndDerivatives=filter  SimscapeFilterOrder=2  InputFilterTimeConstant=whl2rack_filter  UdotUserProvided=0
      settings: AttributesFormatString=|
      | Filter Time Constant
      | %<InputFilterTimeConstant> sec
  Prismatic Rack : sm_lib/Joints/Prismatic Joint  JointMode=Normal  CompositeWrenchDir=FollowerOnBase  CompositeWrenchFrame=BaseFrame  SenseConstraintForce=off  SenseConstraintTorque=off  SenseTotalForce=off  SenseTotalTorque=off  PositionTargetSpecify=on  PositionTargetPriority=Low  PositionTargetValue=0  PositionTargetValueUnits=m  VelocityTargetSpecify=off  VelocityTargetPriority=High  VelocityTargetValue=0  VelocityTargetValueUnits=m/s  EquilibriumPosition=0  EquilibriumPositionUnits=m  SpringStiffness=0  SpringStiffnessUnits=N/m  DampingCoefficient=1e5*0  DampingCoefficientUnits=N/(m/s)  LowerLimitSpecify=off  LowerLimitBound=-1  LowerLimitBoundUnits=m  LowerLimitStiffness=1e6  LowerLimitStiffnessUnits=N/m  LowerLimitDamping=1e3  LowerLimitDampingUnits=N/(m/s)  LowerLimitTransitionRegionWidth=1e-4  LowerLimitTransitionRegionWidthUnits=m  UpperLimitSpecify=off  UpperLimitBound=1  UpperLimitBoundUnits=m  UpperLimitStiffness=1e6  UpperLimitStiffnessUnits=N/m  UpperLimitDamping=1e3  UpperLimitDampingUnits=N/(m/s)  UpperLimitTransitionRegionWidth=1e-4  UpperLimitTransitionRegionWidthUnits=m  TorqueActuationMode=ComputedTorque  MotionActuationMode=InputMotion  SensePosition=on  SenseVelocity=off  SenseAcceleration=off  SenseTorqueForce=on  SenseLowerLimitTorqueForce=off  SenseUpperLimitTorqueForce=off
  Rack : Subsystem  mask{hp_out=hp_out_rack, rack_mass=rack_mass, clr_rack=clr_rack, opc_rack=opc_rack, radius_rack=radius_rack}
      mask prompts: hp_out "HP Track Rod Inboard [xyz] (m)"; rack_mass "Mass (kg)"
      mask init:
      | rack_length = norm(hp_out-hp_out.*[1 -1 1]);
      mask TypeOptions rack_mass: Rack/Mass
      mask TypeOptions clr_rack: Rack/GraphicDiffuseColor
      mask TypeOptions opc_rack: Rack/GraphicOpacity
      mask TypeOptions radius_rack: Rack/CylinderRadius
      mask DialogControl cont_rack Prompt: Rack
      mask DialogControl text_rack_clr Prompt: Color [RGB]
      mask DialogControl text_rack_opc Prompt: Opac. (0-1)
      mask DialogControl text_rack_size Prompt: Size (m)
      mask DialogControl text_rack_rack Prompt: Rack
  Ref to Rack : Subsystem
  Terminator : Terminator
  Terminator1 : Terminator
  Wheel Angle to Rack Displacement : Lookup_n-D  NumberOfTableDimensions=1  BreakpointsForDimension1=whl2rack_whlangle  Table=whl2rack_rackdisp  InternalRulePriority=Speed  RndMeth=Simplest
  rodL : PMIOPort  Side=Right
  ref : PMIOPort  Port=2  Side=Right
  rodR : PMIOPort  Port=3  Side=Right
  Out Bus Element : Outport  VectorParamsAs1DForOutWhenUnconnected=off  PortName=meas  Element=FRack
  Out Bus Element1 : Outport  VectorParamsAs1DForOutWhenUnconnected=off  PortName=meas  Element=xRack
  Out Bus Element2 : Outport  VectorParamsAs1DForOutWhenUnconnected=off  PortName=meas  Element=aWheel
  Out Bus Element3 : Outport  VectorParamsAs1DForOutWhenUnconnected=off  PortName=meas  Element=Driver
  wires:
  Constant/1 -> Out Bus Element2/1
  In Bus Element/1 -> Wheel Angle to Rack Displacement/1
  Wheel Angle to Rack Displacement/1 -> Physical Signal/1
  PS-SL fRack/1 -> Out Bus Element/1
  PS-SL xRack/1 -> Out Bus Element1/1
  In Bus Element2/1 -> Terminator/1
  Body Sensor/1(Body) -> Out Bus Element3/1
  In Bus Element1/1 -> Terminator1/1
  connections:
  rodR/RConn1 -- Rack/LConn2
  rodL/RConn1 -- Body Sensor/LConn1 -- Rack/LConn1
  Prismatic Rack/LConn1 -- Ref to Rack/RConn1
  PS-SL xRack/LConn1 -- Prismatic Rack/RConn2
  Physical Signal/RConn1 -- Prismatic Rack/LConn2
  Rack/RConn1 -- Prismatic Rack/RConn1
  Ref to Rack/LConn1 -- ref/RConn1
  PS-SL fRack/LConn1 -- Prismatic Rack/RConn3

== system Linkage/Susp/Linkage Decoupled/Steer/Rack Driven Shafts ==
  note: Lookup table converts steer angle to rack displacement. For modeling of variable gear ratios.
  note: Shafts and steering wheel are rotated by rack.
  In Bus Element1 : Inport  PortName=DrvBus  Element=aSteerWheel
  In Bus Element : Inport  Port=2  PortName=CtrlBus  Element=aSteerWheel
  Driver : Subsystem  Variant=on  VariantControlMode=label  LabelModeActiveChoice=None  mask{DriverHuman=DriverHuman, VariantLabel=DriverHuman.class.Value}
      mask prompts: DriverHuman "DriverHuman Data (structure)"; VariantLabel "Variant Label"
      mask init:
      | curblk = gcb;
      | 
      | % Set variant for this block 
      | set_param(curblk,'LabelModeActiveChoice',VariantLabel);
      settings: AttributesFormatString=%<LabelModeActiveChoice>
      mask Display: disp(' ')
  HPs : Subsystem
  PS-SL fRack : nesl_utility/PS-Simulink Converter  PhysicalDomain=network_engine_domain  SubClassName=ps_output  LeftPortType=input  RightPortType=output  PseudoPeriodic=off  Frequencies=[]  VectorFormat=1-D array  Unit=N  AffineConversion=off
  PS-SL xRack : nesl_utility/PS-Simulink Converter  PhysicalDomain=network_engine_domain  SubClassName=ps_output  LeftPortType=input  RightPortType=output  PseudoPeriodic=off  Frequencies=[]  VectorFormat=1-D array  Unit=m  AffineConversion=off
  PS-SL xRack1 : nesl_utility/PS-Simulink Converter  PhysicalDomain=network_engine_domain  SubClassName=ps_output  LeftPortType=input  RightPortType=output  PseudoPeriodic=off  Frequencies=[]  VectorFormat=1-D array  Unit=rad  AffineConversion=off
  Physical Signal : nesl_utility/Simulink-PS Converter  PhysicalDomain=network_engine_domain  SubClassName=ps_input  LeftPortType=input  RightPortType=output  PseudoPeriodic=off  Frequencies=[]  NoiseDistribution=none  NoiseParameters=[]  Unit=m  AffineConversion=off  FilteringAndDerivatives=filter  SimscapeFilterOrder=2  InputFilterTimeConstant=steer_filter  UdotUserProvided=0
      settings: AttributesFormatString=|
      | Filter Time Constant
      | %<InputFilterTimeConstant> sec
  Pinion : Subsystem
  Prismatic Rack : sm_lib/Joints/Prismatic Joint  JointMode=Normal  CompositeWrenchDir=FollowerOnBase  CompositeWrenchFrame=BaseFrame  SenseConstraintForce=off  SenseConstraintTorque=off  SenseTotalForce=off  SenseTotalTorque=off  PositionTargetSpecify=on  PositionTargetPriority=High  PositionTargetValue=0  PositionTargetValueUnits=m  VelocityTargetSpecify=off  VelocityTargetPriority=High  VelocityTargetValue=0  VelocityTargetValueUnits=m/s  EquilibriumPosition=0  EquilibriumPositionUnits=m  SpringStiffness=0  SpringStiffnessUnits=N/m  DampingCoefficient=1e5*0  DampingCoefficientUnits=N/(m/s)  LowerLimitSpecify=off  LowerLimitBound=-1  LowerLimitBoundUnits=m  LowerLimitStiffness=1e6  LowerLimitStiffnessUnits=N/m  LowerLimitDamping=1e3  LowerLimitDampingUnits=N/(m/s)  LowerLimitTransitionRegionWidth=1e-4  LowerLimitTransitionRegionWidthUnits=m  UpperLimitSpecify=off  UpperLimitBound=1  UpperLimitBoundUnits=m  UpperLimitStiffness=1e6  UpperLimitStiffnessUnits=N/m  UpperLimitDamping=1e3  UpperLimitDampingUnits=N/(m/s)  UpperLimitTransitionRegionWidth=1e-4  UpperLimitTransitionRegionWidthUnits=m  TorqueActuationMode=ComputedTorque  MotionActuationMode=InputMotion  SensePosition=on  SenseVelocity=off  SenseAcceleration=off  SenseTorqueForce=on  SenseLowerLimitTorqueForce=off  SenseUpperLimitTorqueForce=off
  Rack : Subsystem  mask{hp_out=hp_out_rack, rack_mass=rack_mass, clr_rack=clr_rack, opc_rack=opc_rack, radius_rack=radius_rack}
      mask prompts: hp_out "HP Track Rod Inboard [xyz] (m)"; rack_mass "Mass (kg)"
      mask init:
      | rack_length = norm(hp_out-hp_out.*[1 -1 1]);
      mask TypeOptions rack_mass: Rack/Mass
      mask TypeOptions clr_rack: Rack/GraphicDiffuseColor
      mask TypeOptions opc_rack: Rack/GraphicOpacity
      mask TypeOptions radius_rack: Rack/CylinderRadius
      mask DialogControl cont_rack Prompt: Rack
      mask DialogControl text_rack_clr Prompt: Color [RGB]
      mask DialogControl text_rack_opc Prompt: Opac. (0-1)
      mask DialogControl text_rack_size Prompt: Size (m)
      mask DialogControl text_rack_rack Prompt: Rack
  Rack and Pinion Constraint : sm_lib/Gears and Couplings/Gears/Rack and Pinion Constraint  PinionRadius=rad_pinion  PinionRadiusUnits=m
  Ref to Pinion : Subsystem
  Ref to Rack : Subsystem
  Ref to Wheel : Subsystem
  Revolute Pinion : sm_lib/Joints/Revolute Joint  JointMode=Normal  CompositeWrenchDir=FollowerOnBase  CompositeWrenchFrame=BaseFrame  SenseConstraintForce=off  SenseConstraintTorque=off  SenseTotalForce=off  SenseTotalTorque=off  PositionTargetSpecify=off  PositionTargetPriority=High  PositionTargetValue=0  PositionTargetValueUnits=deg  VelocityTargetSpecify=off  VelocityTargetPriority=High  VelocityTargetValue=0  VelocityTargetValueUnits=deg/s  EquilibriumPosition=0  EquilibriumPositionUnits=deg  SpringStiffness=0  SpringStiffnessUnits=N*m/deg  DampingCoefficient=0  DampingCoefficientUnits=N*m/(deg/s)  LowerLimitSpecify=off  LowerLimitBound=-90  LowerLimitBoundUnits=deg  LowerLimitStiffness=1e4  LowerLimitStiffnessUnits=N*m/deg  LowerLimitDamping=10  LowerLimitDampingUnits=N*m/(deg/s)  LowerLimitTransitionRegionWidth=0.1  LowerLimitTransitionRegionWidthUnits=deg  UpperLimitSpecify=off  UpperLimitBound=90  UpperLimitBoundUnits=deg  UpperLimitStiffness=1e4  UpperLimitStiffnessUnits=N*m/deg  UpperLimitDamping=10  UpperLimitDampingUnits=N*m/(deg/s)  UpperLimitTransitionRegionWidth=0.1  UpperLimitTransitionRegionWidthUnits=deg  TorqueActuationMode=NoTorque  MotionActuationMode=ComputedMotion  SensePosition=off  SenseVelocity=off  SenseAcceleration=off  SenseTorqueForce=off  SenseLowerLimitTorqueForce=off  SenseUpperLimitTorqueForce=off
  Revolute Wheel : sm_lib/Joints/Revolute Joint  JointMode=Normal  CompositeWrenchDir=FollowerOnBase  CompositeWrenchFrame=BaseFrame  SenseConstraintForce=off  SenseConstraintTorque=off  SenseTotalForce=off  SenseTotalTorque=off  PositionTargetSpecify=on  PositionTargetPriority=Low  PositionTargetValue=0  PositionTargetValueUnits=deg  VelocityTargetSpecify=off  VelocityTargetPriority=High  VelocityTargetValue=0  VelocityTargetValueUnits=deg/s  EquilibriumPosition=0  EquilibriumPositionUnits=deg  SpringStiffness=0  SpringStiffnessUnits=N*m/deg  DampingCoefficient=0  DampingCoefficientUnits=N*m/(deg/s)  LowerLimitSpecify=off  LowerLimitBound=-90  LowerLimitBoundUnits=deg  LowerLimitStiffness=1e4  LowerLimitStiffnessUnits=N*m/deg  LowerLimitDamping=10  LowerLimitDampingUnits=N*m/(deg/s)  LowerLimitTransitionRegionWidth=0.1  LowerLimitTransitionRegionWidthUnits=deg  UpperLimitSpecify=off  UpperLimitBound=90  UpperLimitBoundUnits=deg  UpperLimitStiffness=1e4  UpperLimitStiffnessUnits=N*m/deg  UpperLimitDamping=10  UpperLimitDampingUnits=N*m/(deg/s)  UpperLimitTransitionRegionWidth=0.1  UpperLimitTransitionRegionWidthUnits=deg  TorqueActuationMode=NoTorque  MotionActuationMode=ComputedMotion  SensePosition=on  SenseVelocity=off  SenseAcceleration=off  SenseTorqueForce=off  SenseLowerLimitTorqueForce=off  SenseUpperLimitTorqueForce=off
  Shaft Intermediate : Subsystem
  Shaft Lower : Subsystem
  Shaft Upper : Subsystem
  Terminator : Terminator
  Universal Lower : sm_lib/Joints/Universal Joint  JointMode=Normal  CompositeWrenchDir=FollowerOnBase  CompositeWrenchFrame=BaseFrame  SenseConstraintForce=off  SenseConstraintTorque=off  SenseTotalForce=off  SenseTotalTorque=off  RxPositionTargetSpecify=off  RxPositionTargetPriority=High  RxPositionTargetValue=0  RxPositionTargetValueUnits=deg  RxVelocityTargetSpecify=off  RxVelocityTargetPriority=High  RxVelocityTargetValue=0  RxVelocityTargetValueUnits=deg/s  RxEquilibriumPosition=0  RxEquilibriumPositionUnits=deg  RxSpringStiffness=0  RxSpringStiffnessUnits=N*m/deg  RxDampingCoefficient=0  RxDampingCoefficientUnits=N*m/(deg/s)  RxLowerLimitSpecify=off  RxLowerLimitBound=-90  RxLowerLimitBoundUnits=deg  RxLowerLimitStiffness=1e4  RxLowerLimitStiffnessUnits=N*m/deg  RxLowerLimitDamping=10  RxLowerLimitDampingUnits=N*m/(deg/s)  RxLowerLimitTransitionRegionWidth=0.1  RxLowerLimitTransitionRegionWidthUnits=deg  RxUpperLimitSpecify=off  RxUpperLimitBound=90  RxUpperLimitBoundUnits=deg  RxUpperLimitStiffness=1e4  RxUpperLimitStiffnessUnits=N*m/deg  RxUpperLimitDamping=10  RxUpperLimitDampingUnits=N*m/(deg/s)  RxUpperLimitTransitionRegionWidth=0.1  RxUpperLimitTransitionRegionWidthUnits=deg  RxTorqueActuationMode=NoTorque  RxMotionActuationMode=ComputedMotion  RxSensePosition=off  RxSenseVelocity=off  RxSenseAcceleration=off  RxSenseTorqueForce=off  RxSenseLowerLimitTorqueForce=off  RxSenseUpperLimitTorqueForce=off  RyPositionTargetSpecify=off  RyPositionTargetPriority=High  RyPositionTargetValue=0  RyPositionTargetValueUnits=deg  RyVelocityTargetSpecify=off  RyVelocityTargetPriority=High  RyVelocityTargetValue=0  RyVelocityTargetValueUnits=deg/s  RyEquilibriumPosition=0  RyEquilibriumPositionUnits=deg  RySpringStiffness=0  RySpringStiffnessUnits=N*m/deg  RyDampingCoefficient=0  RyDampingCoefficientUnits=N*m/(deg/s)  RyLowerLimitSpecify=off  RyLowerLimitBound=-90  RyLowerLimitBoundUnits=deg  RyLowerLimitStiffness=1e4  RyLowerLimitStiffnessUnits=N*m/deg  RyLowerLimitDamping=10  RyLowerLimitDampingUnits=N*m/(deg/s)  RyLowerLimitTransitionRegionWidth=0.1  RyLowerLimitTransitionRegionWidthUnits=deg  RyUpperLimitSpecify=off  RyUpperLimitBound=90  RyUpperLimitBoundUnits=deg  RyUpperLimitStiffness=1e4  RyUpperLimitStiffnessUnits=N*m/deg  RyUpperLimitDamping=10  RyUpperLimitDampingUnits=N*m/(deg/s)  RyUpperLimitTransitionRegionWidth=0.1  RyUpperLimitTransitionRegionWidthUnits=deg  RyTorqueActuationMode=NoTorque  RyMotionActuationMode=ComputedMotion  RySensePosition=off  RySenseVelocity=off  RySenseAcceleration=off  RySenseTorqueForce=off  RySenseLowerLimitTorqueForce=off  RySenseUpperLimitTorqueForce=off
  Universal Upper : sm_lib/Joints/Universal Joint  JointMode=Normal  CompositeWrenchDir=FollowerOnBase  CompositeWrenchFrame=BaseFrame  SenseConstraintForce=off  SenseConstraintTorque=off  SenseTotalForce=off  SenseTotalTorque=off  RxPositionTargetSpecify=off  RxPositionTargetPriority=High  RxPositionTargetValue=0  RxPositionTargetValueUnits=deg  RxVelocityTargetSpecify=off  RxVelocityTargetPriority=High  RxVelocityTargetValue=0  RxVelocityTargetValueUnits=deg/s  RxEquilibriumPosition=0  RxEquilibriumPositionUnits=deg  RxSpringStiffness=0  RxSpringStiffnessUnits=N*m/deg  RxDampingCoefficient=0  RxDampingCoefficientUnits=N*m/(deg/s)  RxLowerLimitSpecify=off  RxLowerLimitBound=-90  RxLowerLimitBoundUnits=deg  RxLowerLimitStiffness=1e4  RxLowerLimitStiffnessUnits=N*m/deg  RxLowerLimitDamping=10  RxLowerLimitDampingUnits=N*m/(deg/s)  RxLowerLimitTransitionRegionWidth=0.1  RxLowerLimitTransitionRegionWidthUnits=deg  RxUpperLimitSpecify=off  RxUpperLimitBound=90  RxUpperLimitBoundUnits=deg  RxUpperLimitStiffness=1e4  RxUpperLimitStiffnessUnits=N*m/deg  RxUpperLimitDamping=10  RxUpperLimitDampingUnits=N*m/(deg/s)  RxUpperLimitTransitionRegionWidth=0.1  RxUpperLimitTransitionRegionWidthUnits=deg  RxTorqueActuationMode=NoTorque  RxMotionActuationMode=ComputedMotion  RxSensePosition=off  RxSenseVelocity=off  RxSenseAcceleration=off  RxSenseTorqueForce=off  RxSenseLowerLimitTorqueForce=off  RxSenseUpperLimitTorqueForce=off  RyPositionTargetSpecify=off  RyPositionTargetPriority=High  RyPositionTargetValue=0  RyPositionTargetValueUnits=deg  RyVelocityTargetSpecify=off  RyVelocityTargetPriority=High  RyVelocityTargetValue=0  RyVelocityTargetValueUnits=deg/s  RyEquilibriumPosition=0  RyEquilibriumPositionUnits=deg  RySpringStiffness=0  RySpringStiffnessUnits=N*m/deg  RyDampingCoefficient=0  RyDampingCoefficientUnits=N*m/(deg/s)  RyLowerLimitSpecify=off  RyLowerLimitBound=-90  RyLowerLimitBoundUnits=deg  RyLowerLimitStiffness=1e4  RyLowerLimitStiffnessUnits=N*m/deg  RyLowerLimitDamping=10  RyLowerLimitDampingUnits=N*m/(deg/s)  RyLowerLimitTransitionRegionWidth=0.1  RyLowerLimitTransitionRegionWidthUnits=deg  RyUpperLimitSpecify=off  RyUpperLimitBound=90  RyUpperLimitBoundUnits=deg  RyUpperLimitStiffness=1e4  RyUpperLimitStiffnessUnits=N*m/deg  RyUpperLimitDamping=10  RyUpperLimitDampingUnits=N*m/(deg/s)  RyUpperLimitTransitionRegionWidth=0.1  RyUpperLimitTransitionRegionWidthUnits=deg  RyTorqueActuationMode=NoTorque  RyMotionActuationMode=ComputedMotion  RySensePosition=off  RySenseVelocity=off  RySenseAcceleration=off  RySenseTorqueForce=off  RySenseLowerLimitTorqueForce=off  RySenseUpperLimitTorqueForce=off
  Wheel : Subsystem  Variant=on  VariantControlMode=label  LabelModeActiveChoice=FSAE  mask{VariantLabel=Wheel.class.Value}
      mask prompts: VariantLabel "Variant Label"
      mask init:
      | curblk = gcb;
      | 
      | % Set variant for this block 
      | set_param(curblk,'LabelModeActiveChoice',VariantLabel);
      mask Display: disp(' ');
  Wheel Angle to Rack Displacement : Lookup_n-D  NumberOfTableDimensions=1  BreakpointsForDimension1=whl2rack_whlangle  Table=whl2rack_rackdisp  InternalRulePriority=Speed  RndMeth=Simplest
  rodL : PMIOPort  Side=Right
  ref : PMIOPort  Port=2  Side=Right
  rodR : PMIOPort  Port=3  Side=Right
  Out Bus Element : Outport  VectorParamsAs1DForOutWhenUnconnected=off  PortName=meas  Element=FRack
  Out Bus Element1 : Outport  VectorParamsAs1DForOutWhenUnconnected=off  PortName=meas  Element=xRack
  Out Bus Element2 : Outport  VectorParamsAs1DForOutWhenUnconnected=off  PortName=meas  Element=aWheel
  Out Bus Element3 : Outport  VectorParamsAs1DForOutWhenUnconnected=off  PortName=meas  Element=Driver
  wires:
  Driver/1(m) -> Out Bus Element3/1
  Wheel Angle to Rack Displacement/1 -> Physical Signal/1, Driver/1(q)
  PS-SL xRack1/1 -> Out Bus Element2/1
  In Bus Element/1 -> Wheel Angle to Rack Displacement/1
  PS-SL fRack/1 -> Out Bus Element/1
  PS-SL xRack/1 -> Out Bus Element1/1
  In Bus Element1/1 -> Terminator/1
  connections:
  Wheel/RConn2 -- Driver/RConn2
  Driver/RConn1 -- Wheel/RConn1
  Physical Signal/RConn1 -- Prismatic Rack/LConn2
  Prismatic Rack/RConn1 -- Rack/RConn1
  Rack and Pinion Constraint/RConn1 -- Rack/LConn2
  PS-SL xRack/LConn1 -- Prismatic Rack/RConn2
  Ref to Pinion/LConn1 -- ref/RConn1 -- Driver/LConn1 -- Ref to Rack/LConn1 -- HPs/LConn1 -- Ref to Wheel/LConn1
  Rack/LConn1 -- rodL/RConn1
  PS-SL fRack/LConn1 -- Prismatic Rack/RConn3
  Ref to Wheel/RConn1 -- Revolute Wheel/LConn1
  Ref to Pinion/RConn1 -- Revolute Pinion/LConn1
  Ref to Rack/RConn1 -- Prismatic Rack/LConn1
  Universal Lower/LConn1 -- Shaft Lower/LConn1
  Shaft Upper/LConn1 -- Universal Upper/RConn1
  Universal Upper/LConn1 -- Shaft Intermediate/LConn1
  Revolute Wheel/RConn1 -- Shaft Upper/RConn1 -- Wheel/LConn1
  Universal Lower/RConn1 -- Shaft Intermediate/RConn1
  PS-SL xRack1/LConn1 -- Revolute Wheel/RConn2
  rodR/RConn1 -- Rack/LConn3
  Shaft Lower/RConn1 -- Revolute Pinion/RConn1 -- Rack and Pinion Constraint/LConn1 -- Pinion/RConn1
